simulink model "Prj2CDig_continuo_professor"  (R2022b)
settings: Solver=ode45  StartTime=0.0  StopTime=3600  RelTol=1e-6  EnableMultiTasking=on
undefined symbols (not defined in the file): A, B, K, Ki, Kp, L, Nb, PO, Ta, Tp1, Tp2, w0, x1ei, x1i, x2ei, x2i, xii, xs1i, xs2i
settings Model: Creator=Adolfo  LastModifiedBy=adolfo
settings SolverCC: ZeroCrossControl=DisableAll  AlgebraicLoopSolver=TrustRegion
settings DataIOCC: LimitDataPoints=on  MaxDataPoints=25000  SaveFormat=Array  SignalLoggingSaveFormat=ModelDataLogs  ReturnWorkspaceOutputs=off
settings OptimizationCC: BlockReduction=off  BooleanDataType=off  ExpressionDepthLimit=2147483647  InitFltsAndDblsToZero=on  LifeSpan=inf
settings DebuggingCC: SaveWithParameterizedLinksMsg=none  UnderspecifiedInitializationDetection=Classic  MergeDetectMultiDrivingBlocksExec=none  SignalResolutionControl=TryResolveAllWithWarning  MultiTaskDSMMsg=warning  MultiTaskCondExecSysMsg=none  FcnCallInpInsideContextMsg=warning  UnconnectedInputMsg=warning  UnconnectedOutputMsg=warning  UnconnectedLineMsg=warning  StateNameClashWarn=warning  SFUnexpectedBacktrackingDiag=warning  SFNoUnconditionalDefaultTransitionDiag=warning  SFExecutionAtInitializationDiag=none  SFMachineParentedDataDiag=warning  ArithmeticOperatorsInVariantConditions=warning
settings HardwareCC: ProdBitPerPointer=32  ProdBitPerSizeT=32  ProdBitPerPtrDiffT=32  ProdLargestAtomicFloat=None  ProdIntDivRoundTo=Undefined  ProdEndianess=Unspecified  ProdWordSize=32  ProdHWDeviceType=32-bit Generic  TargetUnknown=on
settings ModelReferenceCC: PropagateSignalLabelsOutOfModel=off
settings SFSimCC: SimUseLocalCustomCode=off  CustomCodeUndefinedFunction=UseInterfaceOnly
settings RTWCC: RTWUseLocalCustomCode=off
settings CodeAppCC: StateflowObjectComments=on
settings GRTTargetCC: TargetFcnLib=ansi_tfl_tmw.mat  TargetLangStandard=C89/C90 (ANSI)  CombineOutputUpdateFcns=off  GRTInterface=on
settings ConfigComp: CovMetricSettings=dw  CovSaveCumulativeToWorkspaceVar=on  CovSaveSingleToWorkspaceVar=on

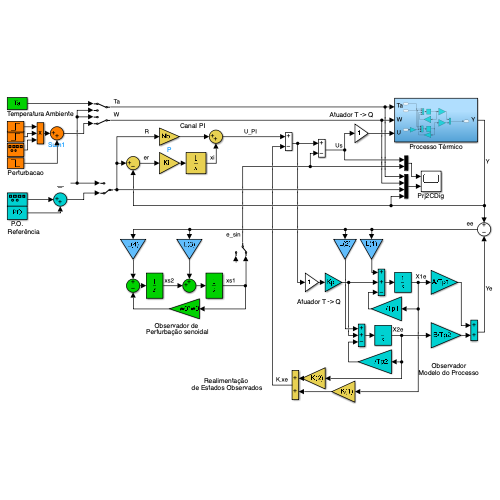
[thumbnail: Simulink's stored preview of the top-level diagram]
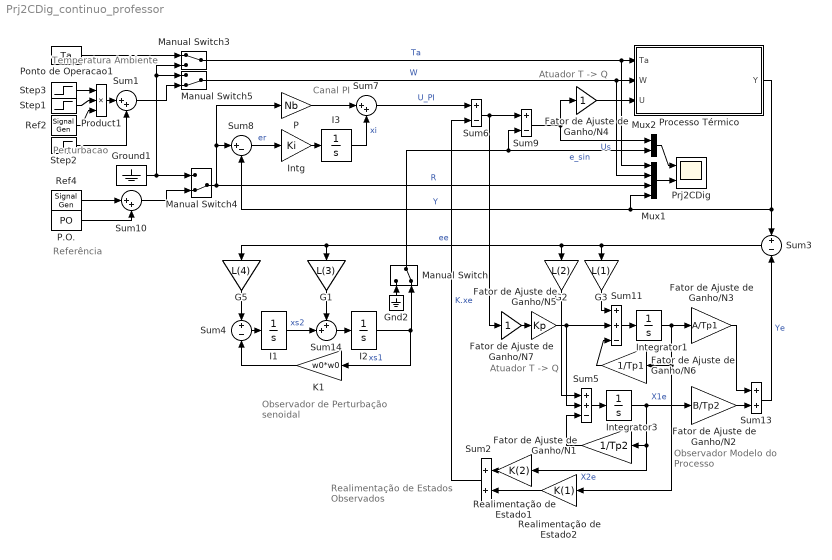
== system Prj2CDig_continuo_professor ==
  note: Temperatura Ambiente
  note: Atuador T -> Q
  note: Referência
  note: Perturbacao
  note: Realimentação
      | de Estados Observados
  note: Observador de
      | Perturbação senoidal
  note: Observador
      | Modelo do Processo
  note: Canal PI
  note: Atuador T -> Q
  Fator de Ajuste de Ganho/N1 : Gain  Gain=1/Tp2  SaturateOnIntegerOverflow=on  OutDataTypeStr=Inherit: Same as input  ParamDataTypeStr=Inherit: Same as input
  Fator de Ajuste de Ganho/N2 : Gain  Gain=B/Tp2  SaturateOnIntegerOverflow=on  OutDataTypeStr=Inherit: Same as input  ParamDataTypeStr=Inherit: Same as input
  Fator de Ajuste de Ganho/N3 : Gain  Gain=A/Tp1  SaturateOnIntegerOverflow=on  OutDataTypeStr=Inherit: Same as input  ParamDataTypeStr=Inherit: Same as input
  Fator de Ajuste de Ganho/N4 : Gain  SaturateOnIntegerOverflow=on  OutDataTypeStr=Inherit: Same as input  ParamDataTypeStr=Inherit: Same as input
  Fator de Ajuste de Ganho/N5 : Gain  Gain=Kp  SaturateOnIntegerOverflow=on  OutDataTypeStr=Inherit: Same as input  ParamDataTypeStr=Inherit: Same as input
  Fator de Ajuste de Ganho/N6 : Gain  Gain=1/Tp1  SaturateOnIntegerOverflow=on  OutDataTypeStr=Inherit: Same as input  ParamDataTypeStr=Inherit: Same as input
  Fator de Ajuste de Ganho/N7 : Gain  SaturateOnIntegerOverflow=on  OutDataTypeStr=Inherit: Same as input  ParamDataTypeStr=Inherit: Same as input
  G1 : Gain  Gain=L(3)  SaturateOnIntegerOverflow=on  OutDataTypeStr=Inherit: Same as input  ParamDataTypeStr=Inherit: Same as input
  G2 : Gain  Gain=L(2)  SaturateOnIntegerOverflow=on  OutDataTypeStr=Inherit: Same as input  ParamDataTypeStr=Inherit: Same as input
  G3 : Gain  Gain=L(1)  SaturateOnIntegerOverflow=on  OutDataTypeStr=Inherit: Same as input  ParamDataTypeStr=Inherit: Same as input
  G5 : Gain  Gain=L(4)  SaturateOnIntegerOverflow=on  OutDataTypeStr=Inherit: Same as input  ParamDataTypeStr=Inherit: Same as input
  Gnd2 : Ground
  Ground1 : Ground
  I1 : Integrator  InitialCondition=xs2i
  I2 : Integrator  InitialCondition=xs1i
  I3 : Integrator  InitialCondition=xii
  Integrator1 : Integrator  InitialCondition=x1ei
  Integrator3 : Integrator  InitialCondition=x2ei
  Intg : Gain  Gain=Ki
  K1 : Gain  Gain=w0*w0  SaturateOnIntegerOverflow=on  OutDataTypeStr=Inherit: Same as input  ParamDataTypeStr=Inherit: Same as input
  Manual Switch : ManualSwitch  CurrentSetting=0
  Manual Switch3 : ManualSwitch
  Manual Switch4 : ManualSwitch  CurrentSetting=0
  Manual Switch5 : ManualSwitch  CurrentSetting=0
  Mux1 : Mux
  Mux2 : Mux  Inputs=2
  P : Gain  Gain=Nb
  P.O. : Constant  Value=PO
  Ponto de Operacao1 : Constant  Value=Ta
  Prj2CDig : Scope  NumInputPorts=2
  Processo Térmico : Subsystem
  Product1 : Product  Inputs=3  RndMeth=Zero
  Realimentação de Estado1 : Gain  Gain=K(2)  SaturateOnIntegerOverflow=on  OutDataTypeStr=Inherit: Same as input  ParamDataTypeStr=Inherit: Same as input
  Realimentação de Estado2 : Gain  Gain=K(1)  SaturateOnIntegerOverflow=on  OutDataTypeStr=Inherit: Same as input  ParamDataTypeStr=Inherit: Same as input
  Ref2 : SignalGenerator  Frequency=w0  Units=rad/sec
  Ref4 : SignalGenerator  WaveForm=square  Amplitude=5  Frequency=.00125
  Step1 : Step  Time=3000  Before=-20  After=0  SampleTime=0
  Step2 : Step  Time=1000  After=-20  SampleTime=0
  Step3 : Step  Time=1800  SampleTime=0
  Sum1 : Sum  Inputs=|++
  Sum10 : Sum  Inputs=|++
  Sum11 : Sum  Inputs=++-
  Sum13 : Sum  InputSameDT=on  SaturateOnIntegerOverflow=on  OutDataTypeStr=Inherit: Same as first input
  Sum14 : Sum  Inputs=++|  InputSameDT=on  SaturateOnIntegerOverflow=on  OutDataTypeStr=Inherit: Same as first input
  Sum2 : Sum
  Sum{3..4,6,9} (4 alike) : Sum  Inputs=+-  InputSameDT=on  SaturateOnIntegerOverflow=on  OutDataTypeStr=Inherit: Same as first input
  Sum5 : Sum  Inputs=++-
  Sum7 : Sum  Inputs=|++
  Sum8 : Sum  Inputs=|+-
  wires:
  Sum9/1 -> Fator de Ajuste de Ganho/N4/1, Mux2/1  "Us"
  P.O./1 -> Sum10/2
  Intg/1 -> I3/1
  Sum8/1 -> Intg/1  "er"
  P/1 -> Sum7/1
  I3/1 -> Sum7/2  "xi"
  Fator de Ajuste de Ganho/N4/1 -> Processo Térmico/3(U)
  Manual Switch5/1 -> Mux1/2, Processo Térmico/2(W)  "W"
  Manual Switch3/1 -> Mux1/1, Processo Térmico/1(Ta)  "Ta"
  Ground1/1 -> Manual Switch3/2, Manual Switch5/1, Manual Switch4/1
  Manual Switch4/1 -> Sum8/1, P/1, Mux1/3  "R"
  Sum1/1 -> Manual Switch5/2
  Ponto de Operacao1/1 -> Manual Switch3/1
  Sum10/1 -> Manual Switch4/2
  Step2/1 -> Sum1/2
  Product1/1 -> Sum1/1
  Processo Térmico/1(Y) -> Sum3/1, Sum8/2, Mux1/4  "Y"
  Fator de Ajuste de Ganho/N1/1 -> Sum5/3
  Integrator1/1 -> Fator de Ajuste de Ganho/N3/1, Fator de Ajuste de Ganho/N6/1, Realimentação de Estado2/1  "X1e"
  Manual Switch/1 -> Mux2/2, Sum9/2  "e_sin"
  Sum2/1 -> Sum6/2  "K.xe"
  Fator de Ajuste de Ganho/N6/1 -> Sum11/3
  Sum3/1 -> G5/1, G1/1, G2/1, G3/1  "ee"
  K1/1 -> Sum4/2
  Realimentação de Estado1/1 -> Sum2/1
  G5/1 -> Sum4/1
  I2/1 -> Manual Switch/2, K1/1  "xs1"
  Sum11/1 -> Integrator1/1
  Fator de Ajuste de Ganho/N2/1 -> Sum13/2
  Realimentação de Estado2/1 -> Sum2/2
  Sum5/1 -> Integrator3/1
  G3/1 -> Sum11/1
  Integrator3/1 -> Fator de Ajuste de Ganho/N2/1, Fator de Ajuste de Ganho/N1/1, Realimentação de Estado1/1  "X2e"
  Sum4/1 -> I1/1
  G2/1 -> Sum5/1
  Sum7/1 -> Sum6/1  "U_PI"
  Fator de Ajuste de Ganho/N5/1 -> Sum5/2, Sum11/2
  Sum14/1 -> I2/1
  I1/1 -> Sum14/2  "xs2"
  G1/1 -> Sum14/1
  Sum13/1 -> Sum3/2  "Ye"
  Fator de Ajuste de Ganho/N3/1 -> Sum13/1
  Sum6/1 -> Sum9/1, Fator de Ajuste de Ganho/N7/1
  Ref4/1 -> Sum10/1
  Gnd2/1 -> Manual Switch/1
  Mux1/1 -> Prj2CDig/2
  Fator de Ajuste de Ganho/N7/1 -> Fator de Ajuste de Ganho/N5/1
  Mux2/1 -> Prj2CDig/1
  Ref2/1 -> Product1/3
  Step1/1 -> Product1/2
  Step3/1 -> Product1/1

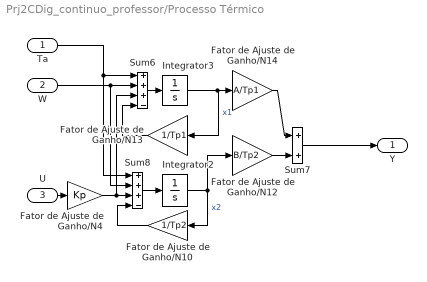
== system Prj2CDig_continuo_professor/Processo Térmico ==
  Ta : Inport
  W : Inport  Port=2
  U : Inport  Port=3
  Fator de Ajuste de Ganho/N10 : Gain  Gain=1/Tp2  SaturateOnIntegerOverflow=on  OutDataTypeStr=Inherit: Same as input  ParamDataTypeStr=Inherit: Same as input
  Fator de Ajuste de Ganho/N12 : Gain  Gain=B/Tp2  SaturateOnIntegerOverflow=on  OutDataTypeStr=Inherit: Same as input  ParamDataTypeStr=Inherit: Same as input
  Fator de Ajuste de Ganho/N13 : Gain  Gain=1/Tp1  SaturateOnIntegerOverflow=on  OutDataTypeStr=Inherit: Same as input  ParamDataTypeStr=Inherit: Same as input
  Fator de Ajuste de Ganho/N14 : Gain  Gain=A/Tp1  SaturateOnIntegerOverflow=on  OutDataTypeStr=Inherit: Same as input  ParamDataTypeStr=Inherit: Same as input
  Fator de Ajuste de Ganho/N4 : Gain  Gain=Kp  SaturateOnIntegerOverflow=on  OutDataTypeStr=Inherit: Same as input  ParamDataTypeStr=Inherit: Same as input
  Integrator2 : Integrator  InitialCondition=x2i
  Integrator3 : Integrator  InitialCondition=x1i
  Sum6 : Sum  Inputs=+++-
  Sum7 : Sum  InputSameDT=on  SaturateOnIntegerOverflow=on  OutDataTypeStr=Inherit: Same as first input
  Sum8 : Sum  Inputs=+++-
  Y : Outport
  wires:
  Fator de Ajuste de Ganho/N12/1 -> Sum7/2
  Fator de Ajuste de Ganho/N13/1 -> Sum6/4
  Sum8/1 -> Integrator2/1
  Sum6/1 -> Integrator3/1
  Fator de Ajuste de Ganho/N10/1 -> Sum8/4
  U/1 -> Fator de Ajuste de Ganho/N4/1
  Fator de Ajuste de Ganho/N14/1 -> Sum7/1
  Integrator3/1 -> Fator de Ajuste de Ganho/N14/1, Fator de Ajuste de Ganho/N13/1  "x1"
  Integrator2/1 -> Fator de Ajuste de Ganho/N12/1, Fator de Ajuste de Ganho/N10/1  "x2"
  Ta/1 -> Sum8/1, Sum6/1
  Fator de Ajuste de Ganho/N4/1 -> Sum6/3, Sum8/3
  W/1 -> Sum8/2, Sum6/2
  Sum7/1 -> Y/1
